simulink model "SPdyn"  (R2021b)
settings: Solver=VariableStepAuto  StartTime=0.0  StopTime=10.0  MaxStep=0.005  RelTol=1e-3
values from neighbouring files (symbols this model uses):
  g = 32.17405    [SingleDOF.m]    (also in layer1atm.m; mainSimple.m = 32.174; simio.m = [dx(Index.EOM(1:6)); delta(:)-f; -delta(:)-f ])
  K_lon_hinf = pss(K_lon_hinfs,Domain)    [SingleDOF.m]    (also in main.m; mainSimple.m)
  LTI_lon = ss(A,B,C,D)    [Dorobantu.m]    (also in mainLinear.m = GTM_lon(:,:,i,j,k); newmain.m = GTM_lon(:,:,i,j,k))
libraries: simulink_extras x4
settings Model: Creator=jihoo  LastModifiedBy=jihoo

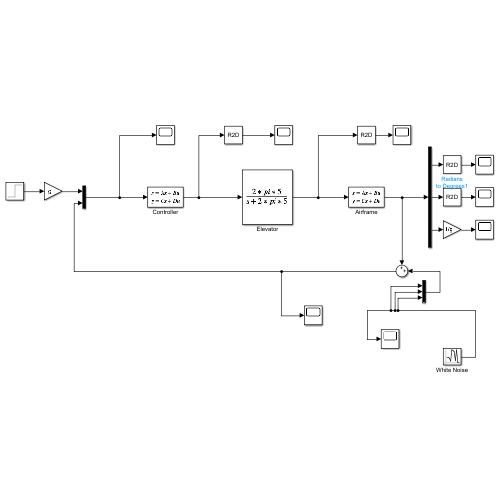
[thumbnail: Simulink's stored preview of the top-level diagram]
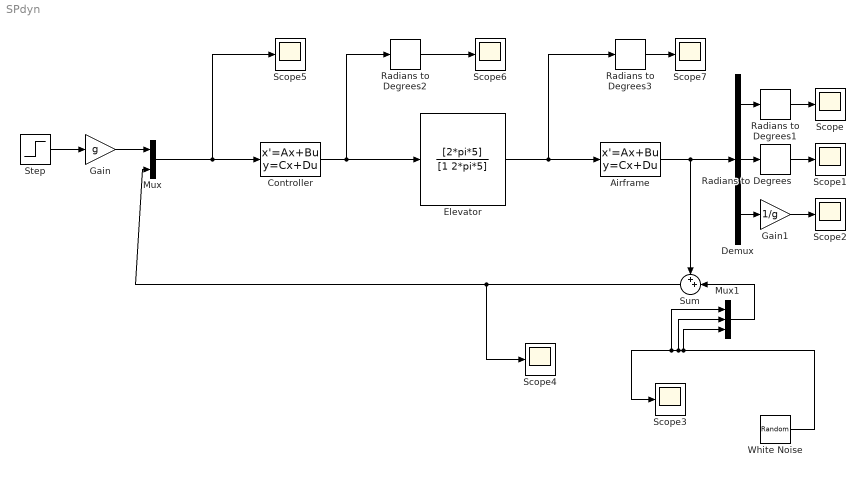
== system SPdyn ==
  Airframe : StateSpace  A=LTI_lon.A  B=LTI_lon.B  C=LTI_lon.C  D=LTI_lon.D  InitialCondition=0
  Controller : StateSpace  A=K_lon_hinf.A  B=K_lon_hinf.B  C=K_lon_hinf.C  D=K_lon_hinf.D  InitialCondition=0
  Demux : Demux  Outputs=3
  Elevator : TransferFcn  Numerator=[2*pi*5]  Denominator=[1 2*pi*5]
  Gain : Gain  Gain=g
  Gain1 : Gain  Gain=1/g
  Mux : Mux  Inputs=[1 3]
  Mux1 : Mux  Inputs=3
  Radians to Degrees{,1..3} (4 alike) : simulink_extras/Transformations/Radians to Degrees
  Scope{,1..7} (8 alike) : Scope
  Step : Step  Time=0  SampleTime=0
  Sum : Sum  Inputs=++|
  White Noise : RandomNumber  Mean=1000  Variance=1000  Seed=round(300*rand(1))  SampleTime=1/200
  wires:
  Mux/1 -> Scope5/1, Controller/1
  Airframe/1 -> Demux/1, Sum/1
  Demux/1 -> Radians to Degrees1/1
  Demux/2 -> Radians to Degrees/1
  Demux/3 -> Gain1/1
  Step/1 -> Gain/1
  Gain/1 -> Mux/1
  Gain1/1 -> Scope2/1
  Radians to Degrees/1 -> Scope1/1
  Radians to Degrees1/1 -> Scope/1
  Controller/1 -> Radians to Degrees2/1, Elevator/1
  Elevator/1 -> Radians to Degrees3/1, Airframe/1
  White Noise/1 -> Mux1/3, Mux1/2, Mux1/1, Scope3/1
  Sum/1 -> Scope4/1, Mux/2
  Radians to Degrees2/1 -> Scope6/1
  Radians to Degrees3/1 -> Scope7/1
  Mux1/1 -> Sum/2
